simulink model "ecu_muclose"  (R2026a)
settings: Solver=FixedStepDiscrete  StopTime=10  FixedStep=0.001  SampleTimeConstraint=STIndependent
Description:
  | Closed-valve duty on the learned coil. Source of truth for firmware/gen/ecu_muclose.
settings Model: Creator=jj1001000  LastModifiedBy=jj1001000
settings OptimizationCC: DefaultUnderspecifiedDataType=single
settings DebuggingCC: ParameterPrecisionLossMsg=none
settings HardwareCC: ProdLargestAtomicInteger=Long  ProdLargestAtomicFloat=Double  ProdHWDeviceType=ARM Compatible->ARM Cortex-M
settings RTWCC: SystemTargetFile=ert.tlc  GenCodeOnly=on  Description=Embedded Coder
settings ERTTargetCC: UtilityFuncGeneration=Shared location  IncludeMdlTerminateFcn=off  CodeInterfacePackaging=Reusable function  SupportNonFinite=off

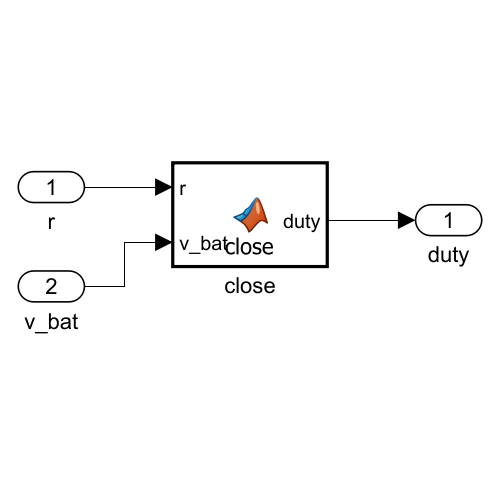
[thumbnail: Simulink's stored preview of the top-level diagram]
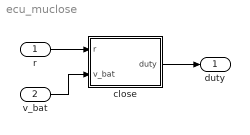
== system ecu_muclose ==
  r : Inport  OutDataTypeStr=single
  v_bat : Inport  Port=2  OutDataTypeStr=single
  close : MATLAB Function  TreatAsAtomicUnit=on
  duty : Outport  OutDataTypeStr=single
  wires:
  close/1(duty) -> duty/1
  v_bat/1 -> close/2(v_bat)
  r/1 -> close/1(r)

== matlab function ecu_muclose/close ==
  data: r input single; duty output single; v_bat input single
function duty = close(r, v_bat)
%#codegen
rc = r;
if rc < single(1.85000002)
    rc = single(1.85000002);
elseif rc > single(6.90999985)
    rc = single(6.90999985);
end
c = single(1) * (rc / single(3.75));
if v_bat >= single(6) && v_bat <= single(18)
    vb = v_bat;
else
    vb = single(13.5);
end
duty = c * (single(6.75) / vb);
if duty < single(0)
    duty = single(0);
elseif duty > single(1)
    duty = single(1);
end
